simulink model "fox_twin_replay"  (R2025b)
settings: Solver=FixedStepDiscrete  StartTime=0.0  StopTime=1.96  FixedStep=0.001  RelTol=1e-3
model workspace (MAT data in the model file):
  actuators = [74.5 74.5 74.5 74.5 74.5 74.5 74.5 74.5 74.5 74.5 74.5 74.5 ... (5883 elements, 1961x3)]
  encoderParameters = [7.523; 1.00345584192; 0.05; 2e-05; 0.02; 53]
  fieldSegments = [1500  -1500  1500  1500; 1500  1500  -1500  1500; -1500  1500  -1500  -1500; -1500  -1500  1500  -1500; 500  -500  500  500; 500  500  -500  500; -500  500  -500  -500; -500  -500  500  -500; -1500  -89.2  -1500  -69.2; -1500  -69.2  -1300  -69.2; -1300  -69.2  -1300  -89.2; -1300  -89.2  -1500  -89.2; -1500  194.8  -1500  214.8; -1500  214.8  -1300  214.8; -1300  214.8  -1300  194.8; -1300  194.8  -1500  194.8; 1075  -25  1125  -25; 1125  -25  1125  25; 1125  25  1075  25; 1075  25  1075  -25; 475  1075  525  1075; 525  1075  525  1125; 525  1125  475  1125; 475  1125  475  1075; -525  1075  -475  1075; -475  1075  -475  1125; -475  1125  -525  1125; -525  1125  -525  1075; -525  -925  -475  -925; -475  -925  -475  -875; -475  -875  -525  -875; -525  -875  -525  -925; -925  475  -875  475; -875  475  -875  525; -875  525  -925  525; -925  525  -925  475; -925  -525  -875  -525; -875  -525  -875  -475; -875  -475  -925  -475; -925  -475  -925  -525]
  initialState = [-1000; 0; 0; 0; 90; 90; 0; 0; 90; -8.66666666667; 0; 0]
  plantParameters = [156; 1; 0.5; 600; 1.5; 0.1; 74.5; 57; 46.2; 53; 53; 22.9; 600; 4700; 5000; 0.06; 1000; 1; 6; 37.6; 6.51; 53; 0.12; 0.091; 0.28; 1200; 4316; 1; 0.06; 0.9; 113; 2400; 2750; 4; 4; 0; 0; 13.5; 8.7; 28.5; 18.2; 72.5; 53; 0; 0; 13.5; 7.6; 28.5; 15.6; 71.5; 53]
  sampleTime = 0.001
  sensorMounts = [-35.2  110.6  270  1300; 35.2  110.6  90  1300; 0  -19.6  180  1300; 0  141.4  0  4000]
settings Model: Creator=runner  LastModifiedBy=runner

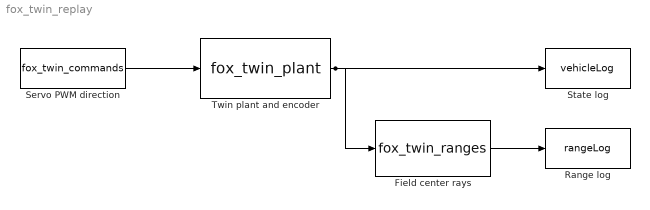
== system fox_twin_replay ==
  Field center rays : M-S-Function  FunctionName=fox_twin_ranges  Parameters=fieldSegments, sensorMounts
  Range log : ToWorkspace  VariableName=rangeLog  SaveFormat=Structure With Time  SampleTime=-1
  Servo PWM direction : M-S-Function  FunctionName=fox_twin_commands  Parameters=actuators, sampleTime
  State log : ToWorkspace  VariableName=vehicleLog  SaveFormat=Structure With Time  SampleTime=-1
  Twin plant and encoder : M-S-Function  FunctionName=fox_twin_plant  Parameters=plantParameters, encoderParameters, initialState, sampleTime
  wires:
  Servo PWM direction/1 -> Twin plant and encoder/1
  Twin plant and encoder/1 -> State log/1, Field center rays/1
  Field center rays/1 -> Range log/1
